simulink model "hysteretic_controller_Buck_converter_A01"  (R2025b)
settings: Solver=ode15s  StartTime=0.0  StopTime=0.1  FixedStep=Ts  RelTol=1e-3
values from neighbouring files (symbols this model uses):
  Ki = 100    [buck_converter_parameters_A01.m]    (also in hysteretic_controller_simu_A01.m = 1000)
  Kp = 80    [buck_converter_parameters_A01.m]    (also in hysteretic_controller_simu_A01.m = 1)
  Vhys = 0.01    [buck_converter_parameters_A01.m]    (also in hysteretic_controller_simu_A01.m = 0.2; latched_hysteretic_circuit_A01.m = 0.5)
libraries: spsSeriesRLCBranchLib x3, spsCurrentMeasurementLib x2, spsDCVoltageSourceLib x1, spsDiodeLib x1, spsMosfetLib x1, spsVoltageMeasurementLib x1, sps_lib x1
settings Model: Creator=arif  LastModifiedBy=arif
settings SolverCC: ZeroCrossAlgorithm=Adaptive
settings DebuggingCC: MaskedZcDiagnostic=none  IgnoredZcDiagnostic=none

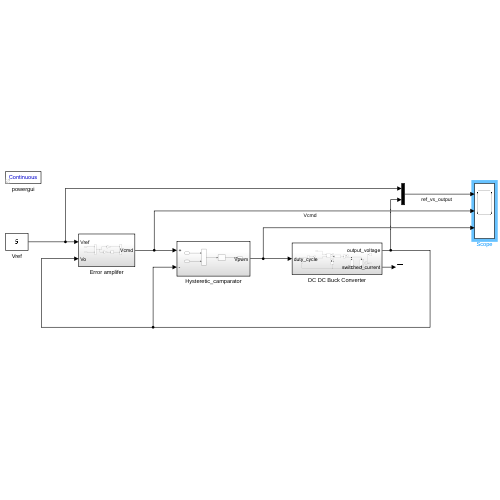
[thumbnail: Simulink's stored preview of the top-level diagram]
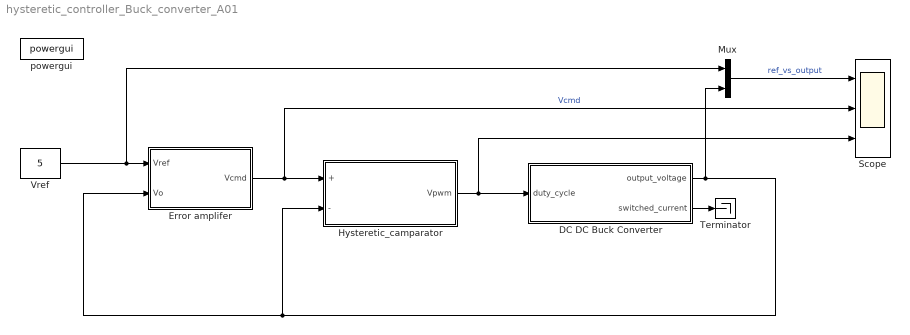
== system hysteretic_controller_Buck_converter_A01 ==
  DC DC Buck Converter : Subsystem
  Error amplifer : Subsystem
  Hysteretic_camparator : Subsystem
  Mux : Mux  Inputs=2
  Scope : Scope  NumInputPorts=3
      settings: ActiveDisplayYMinimum=-1.8005718240674735  ActiveDisplayYMaximum=16.213546164614826
  Terminator : Terminator
  Vref : Constant  Value=5
  powergui : sps_lib/powergui  Priority=1  SimulationMode=Continuous  SampleTime=50e-6  frequency=60  Iterations=50  frequencyindice=0  Pbase=100e6  ErrMax=1e-4  UnitsV=kV  UnitsW=MW  buscounter=0  FunctionMessages=off  echomessages=off  EnableUseOfTLC=off  CurrentSourceSwitches=off  DisableSnubberDevices=off  DisableRonSwitches=off  DisableVfSwitches=off  DisplayEquations=off  AutomaticDiscreteSolvers=off  SolverType=Tustin/Backward Euler (TBE)  Interpol=off  ExternalGateDelay=off  methode=off  Ts=100  x0status=blocks  SPID=on  SwTol=0  HookPort=off  NonlinearTolerance=1e-4  nMaxIteration=100  ContinueOnMaxIteration=off  RestoreLinks=warning  ResistiveCurrentMeasurement=off  Frange=[0:2:500]  Ylog=off  Xlog=on  ShowGrid=off  save=off  variable=ZData  structure=0  ZoomFFT=off  StartTime=0.0  cycles=1  DisplayStyle=1  fundamental=60  FreqAxis=off  MaxFrequency=1000  frequencyindicesteady=1  RmsSteady=1  display=off
  wires:
  DC DC Buck Converter/2(switched_current) -> Terminator/1
  DC DC Buck Converter/1(output_voltage) -> Mux/2, Error amplifer/2(Vo), Hysteretic_camparator/2(-)
  Hysteretic_camparator/1(Vpwm) -> Scope/3, DC DC Buck Converter/1(duty_cycle)
  Vref/1 -> Mux/1, Error amplifer/1(Vref)
  Error amplifer/1(Vcmd) -> Scope/2, Hysteretic_camparator/1(+)  "Vcmd"
  Mux/1 -> Scope/1  "ref_vs_output"

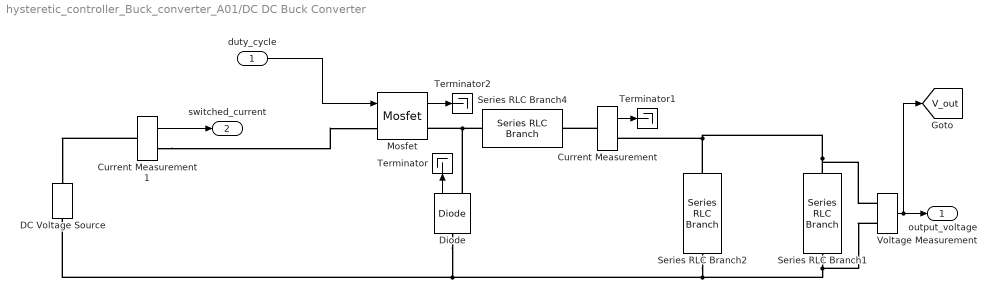
== system hysteretic_controller_Buck_converter_A01/DC DC Buck Converter ==
  duty_cycle : Inport
  Current Measurement : spsCurrentMeasurementLib/Current Measurement  PhasorSimulation=off  OutputType=Complex  PSBequivalent=0
  Current Measurement1 : spsCurrentMeasurementLib/Current Measurement  PhasorSimulation=off  OutputType=Complex  PSBequivalent=0
  DC Voltage Source : spsDCVoltageSourceLib/DC Voltage Source  Amplitude=28  Measurements=None
  Diode : spsDiodeLib/Diode  Ron=0.001  Lon=0  Vf=0.8  IC=0  UseSnubber=0  Rs=500  Cs=250e-9  Measurements=on
  Mosfet : spsMosfetLib/Mosfet  Ron=0.1  Lon=0  Rd=0.01  Vfd=0  IC=0  Rs=1e5  Cs=inf  Measurements=on
  Series RLC Branch1 : spsSeriesRLCBranchLib/Series RLC Branch  LConnTagsString=__new0  RConnTagsString=__new0  BranchType=R  Resistance=3  Inductance=1e-3  SetiL0=off  InitialCurrent=0  Capacitance=1e-6  Setx0=off  InitialVoltage=0  Measurements=None
  Series RLC Branch2 : spsSeriesRLCBranchLib/Series RLC Branch  LConnTagsString=__new0  RConnTagsString=__new0  BranchType=C  Resistance=10  Inductance=1e-3  SetiL0=off  InitialCurrent=0  Capacitance=500e-6  Setx0=off  InitialVoltage=0  Measurements=None
  Series RLC Branch4 : spsSeriesRLCBranchLib/Series RLC Branch  LConnTagsString=__new0  RConnTagsString=__new0  BranchType=L  Resistance=10  Inductance=50e-6  SetiL0=off  InitialCurrent=0  Capacitance=1e-6  Setx0=off  InitialVoltage=0  Measurements=None
  Terminator : Terminator
  Terminator1 : Terminator
  Terminator2 : Terminator
  Voltage Measurement : spsVoltageMeasurementLib/Voltage Measurement  PhasorSimulation=off  OutputType=Complex  PSBequivalent=0
  output_voltage : Outport
  switched_current : Outport  Port=2
  tag scope: V_out=global
  wires:
  Current Measurement/1 -> Terminator1/1
  Diode/1 -> Terminator/1
  duty_cycle/1 -> Mosfet/1
  Mosfet/1 -> Terminator2/1
  Current Measurement1/1 -> switched_current/1
  Voltage Measurement/1 -> [V_out], output_voltage/1
  connections:
  Current Measurement1/RConn1 -- Mosfet/LConn1
  Current Measurement1/LConn1 -- DC Voltage Source/RConn1
  Mosfet/RConn1 -- Series RLC Branch4/LConn1 -- Diode/RConn1
  DC Voltage Source/LConn1 -- Series RLC Branch1/RConn1 -- Voltage Measurement/LConn2 -- Series RLC Branch2/RConn1 -- Diode/LConn1
  Series RLC Branch1/LConn1 -- Series RLC Branch2/LConn1 -- Current Measurement/RConn1 -- Voltage Measurement/LConn1
  Current Measurement/LConn1 -- Series RLC Branch4/RConn1

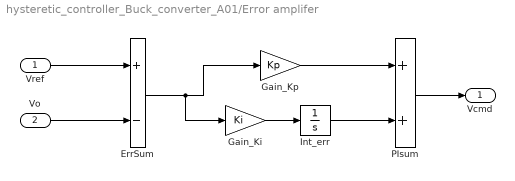
== system hysteretic_controller_Buck_converter_A01/Error amplifer ==
  Vref : Inport
  Vo : Inport  Port=2
  ErrSum : Sum  Inputs=+-
  Gain_Ki : Gain  Gain=Ki
  Gain_Kp : Gain  Gain=Kp
  Int_err : Integrator
  PIsum : Sum
  Vcmd : Outport
  wires:
  PIsum/1 -> Vcmd/1
  Gain_Kp/1 -> PIsum/1
  Int_err/1 -> PIsum/2
  Gain_Ki/1 -> Int_err/1
  ErrSum/1 -> Gain_Kp/1, Gain_Ki/1
  Vo/1 -> ErrSum/2
  Vref/1 -> ErrSum/1

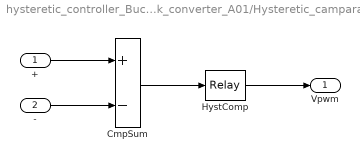
== system hysteretic_controller_Buck_converter_A01/Hysteretic_camparator ==
  + : Inport
  - : Inport  Port=2
  CmpSum : Sum  Inputs=+-
  HystComp : Relay  OnSwitchValue=Vhys/2  OffSwitchValue=-Vhys/2
  Vpwm : Outport
  wires:
  CmpSum/1 -> HystComp/1
  HystComp/1 -> Vpwm/1
  -/1 -> CmpSum/2
  +/1 -> CmpSum/1
